simulink model "CLLCTestHarnessPlant"  (R2026a)
settings: Solver=ode23t  StopTime=5e-3  FixedStep=1e-4  MaxStep=1e-6  AbsTol=1e-3
PreLoadFcn:
  | CLLCConverterDefaultInputParameters;
undefined symbols (not defined in the file or in its folder): CLLCCompensator, CLLCController, CLLCDesign, DiscIntNeverNeededParam
libraries: fl_lib x46, nesl_utility x45, ee_lib x35
(part 4 of 4)

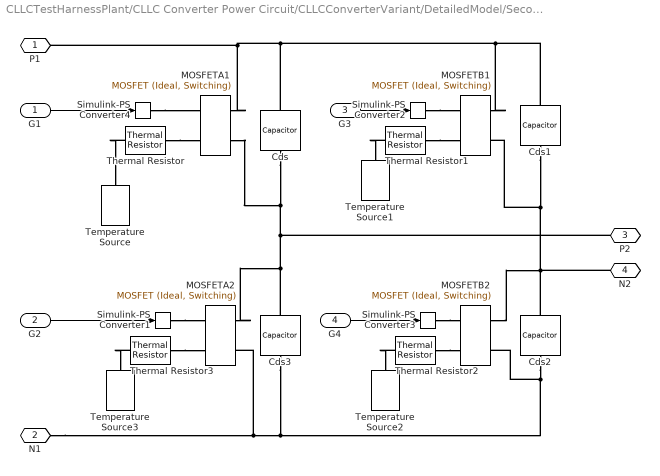
== system CLLCTestHarnessPlant/CLLC Converter Power Circuit/CLLCConverterVariant/DetailedModel/Secondary Converter/Secondary Converter Full Bridge/Ideal MOSFET with Thermal ==
  G1 : Inport
  G2 : Inport  Port=2
  G3 : Inport  Port=3
  G4 : Inport  Port=4
  Cds{,1..3} (4 alike) : fl_lib/Electrical/Electrical Elements/Capacitor  c=SecondaryCparasitic F  r=0.05 Ohm  g=1e-5 1/Ohm  i_specify=off  i_priority=None  i=0 A  i_nominal_specify=off  i_nominal_value=1  i_nominal_unit=A  v_specify=off  v_priority=None  v=0 V  v_nominal_specify=off  v_nominal_value=1  v_nominal_unit=V  vc_specify=on  vc_priority=None  vc=0 V  vc_nominal_specify=off  vc_nominal_value=1  vc_nominal_unit=V
  MOSFETA1 : ee_lib/Semiconductors & Converters/MOSFET (Ideal, Switching)  PartSpecification="{\"CollectionId\":\"MW.SimscapeElectrical\",\"CollectionVersion\":\"1.0.0\",\"DatasetId\":\"Wolfspeed|C3M0015065D|simscape.electrical.mosfetIdealSwitching\",\"DisplayName\":\"Wolfspeed:C3M0015065D\"}"  port_option=ee.enum.controlport.ps  Rds=0.015 % Datasheet derived Ohm  Goff=1.53846153846154e-09 % Datasheet derived S  Vth=2.3 % Datasheet derived V  diode_param=ee.enum.semiconductors.protectionDiode.nodynamics  diode_Vf=1.96 % Datasheet derived V  diode_Ron=0.007 % Wolfspeed XML derived Ohm  diode_Goff=1e-05 % Library default S  diode_C=50e-9 % Parameter not set F  diode_iRM=-235 % Parameter not set A  diode_iF=300 % Parameter not set A  diode_idot=-50 % Parameter not set A/us  diode_trr_param=ee.enum.converters.diodeReverseParam.trr_factor  diode_trr_factor=3 % Parameter not set  diode_trr=15 % Parameter not set us  diode_Qrr=1500 % Parameter not set s*uA  ids_specify=off  ids_priority=None  ids=0 A  ids_nominal_specify=off  ids_nominal_value=1  ids_nominal_unit=A  vds_specify=off  vds_priority=None  vds=0 V  vds_nominal_specify=off  vds_nominal_value=1  vds_nominal_unit=V  vgs_specify=off  vgs_priority=None  vgs=0 V  vgs_nominal_specify=off  vgs_nominal_value=1  vgs_nominal_unit=V  thermal_loss_option=ee.enum.converters.thermalLossOption.tabulated2d  Von_data=[-2.66 -2.44 -1.95 -1.414 -0.78 -0.41 -0.165 -0.082 -0.0343 0 0.037 0.078 0.179 0.43 0.83 1.68 2.597 3.5358 4.01;-2.83 -2.54 -1.975 -1.397 -0.75 -0.38 -0.155 -0.08 -0.03 0 0.034 0.067 0.16 0.39 0.76 1.549 2.4 3.26 3.72;-4.517 -4 -2.934 -1.965 -1 -0.51 -0.2048 -0.1018 -0.041 0 0.042 0.085 0.2 0.496 0.997 2.035 3.12 4.4 5.045;-5 -4.4 -3.2274 -2.1615 -1.1 -0.561 -0.22528 -0.11198 -0.0451 0 0.0462 0.0935 0.22 0.5456 1.0967 2.2385 3.432 4.84 5.5495] % Wolfspeed XML derived V  Tj=[-40 25 175 900] % Wolfspeed XML derived degC  Iout_data=[-225 -200 -150 -100 -50 -25 -10 -5 -2 0 2 5 10 25 50 100 150 200 225] % Wolfspeed XML derived A  tabulateWithVds=true  Eon_data=[0 0.000296720706 0.000619737448 0.001060530449 0.001624353636 0.002289518971 0.003055101185 0.003909744423 0.004857655737;0 0.000278295464 0.000568760601 0.000943163001 0.001425114545 0.001997455958 0.002650659932 0.003379733973 0.004171975428;0 0.000279540051 0.000560708357 0.000946039081 0.001433453185 0.002004053998 0.002654023251 0.00337272687 0.004157099722;0 0.000287359198 0.000590152745 0.001002040365 0.001504786569 0.002087057353 0.002740975089 0.003462716804 0.004216675388;0 0.000330463078 0.000678675657 0.00115234642 0.001730504555 0.002400115956 0.003152121352 0.003982124325 0.004849176696] % Wolfspeed XML derived J  Eoff_data=[0 4.1760829e-05 0.000185261132 0.00041711825 0.000737680365 0.001120556246 0.001567378167 0.002077858914 0.002638540549;0 3.7063976e-05 0.000164368774 0.000376314901 0.000674169231 0.001014162086 0.001431179744 0.001884719714 0.002400774934;0 4.0061697e-05 0.000173404947 0.000400371607 0.000703518786 0.001068777044 0.001494839984 0.001971248404 0.002508087918;0 4.0265683e-05 0.000184357503 0.000417637115 0.000741131352 0.001127026128 0.001573263077 0.002066583681 0.002614125351;0 4.6305536e-05 0.000212011129 0.000480282682 0.000852301054 0.001296080048 0.001809252539 0.002376571234 0.003006244154] % Wolfspeed XML derived J  Eon_data_3D=reshape([0;0;0;0;0;0;0;0;0;0;0;0;0;0;0;0;0;0;0;0;0;0;0;0;0;0;0;0;0;0;0;0;0;0;0;0;0;0;0;0;0;0;0;0;0;0;0;0;0;0;0;0;0;0;0;0;0;0;0;0;0;0;0;0;0;0;0;0;0;0;0;0;0;0;0;0;0;0;0;0;0;0;0;0;0;0;0;0;0;0;0;0;0;0;0;0.000296720706;0.000278295464;0.000279540051;0.000287359198;0.000330463078;0.000619737448;0.000568760601;0.000560708357;0.000590152745;0.000678675657;0.001060530449;0.000943163001;0.000946039081;0.001002040365;0.00115234642;0.001624353636;0.001425114545;0.001433453185;0.001504786569;0.001730504555;0.002289518971;0.001997455958;0.002004053998;0.002087057353;0.002400115956;0.003055101185;0.002650659932;0.002654023251;0.002740975089;0.003152121352;0.003909744423;0.003379733973;0.00337272687;0.003462716804;0.003982124325;0.004857655737;0.004171975428;0.004157099722;0.004216675388;0.004849176696],[5 9 3]) % Wolfspeed XML derived J  Eoff_data_3D=reshape([0;0;0;0;0;0;0;0;0;0;0;0;0;0;0;0;0;0;0;0;0;0;0;0;0;0;0;0;0;0;0;0;0;0;0;0;0;0;0;0;0;0;0;0;0;0;0;0;0;0;0;0;0;0;0;0;0;0;0;0;0;0;0;0;0;0;0;0;0;0;0;0;0;0;0;0;0;0;0;0;0;0;0;0;0;0;0;0;0;0;0;0;0;0;0;4.1760829e-05;3.7063976e-05;4.0061697e-05;4.0265683e-05;4.6305536e-05;0.000185261132;0.000164368774;0.000173404947;0.000184357503;0.000212011129;0.00041711825;0.000376314901;0.000400371607;0.000417637115;0.000480282682;0.000737680365;0.000674169231;0.000703518786;0.000741131352;0.000852301054;0.001120556246;0.001014162086;0.001068777044;0.001127026128;0.001296080048;0.001567378167;0.001431179744;0.001494839984;0.001573263077;0.001809252539;0.002077858914;0.001884719714;0.001971248404;0.002066583681;0.002376571234;0.002638540549;0.002400774934;0.002508087918;0.002614125351;0.003006244154],[5 9 3]) % Wolfspeed XML derived J  Tj_loss=[25 75 125 175 900] % Wolfspeed XML derived degC  Iout_data_loss=[0 13.2 26 38.8 50.8 62.8 74.8 86 97.2] % Wolfspeed XML derived A  Vds_loss=[-10 0 400] % Wolfspeed XML derived V  Eon_scalar=22.86e-3 % Parameter not set J  Eoff_scalar=17.14e-3 % Parameter not set J  Voff=300 % Parameter not set V  Iout_scalar=600 % Parameter not set A  useCurrentFromPreviousCycle=false  useVoltageFromPreviousCycle=false  diodeModelType=ee.enum.converters.diodeModelType.tabulated  diodeTableType=ee.enum.diode.tableType.VfMat  diode_ReverseIVType=ee.enum.diode.diodeReverseIV.constant  diode_IfMat=[.07, .12, .19, 1.75, 4.24, 7.32, 11.2; .16, .3, .72, 2.14, 4.02, 6.35, 9.12] % Parameter not set A  diode_VfMat=[0 2.87 3.94 4.34 5.07 5.76 6.58 7.12 7.53 7.697;0 2.68 3.54 3.9 4.55 5.26 6.12 6.72 7.18 7.38;0 2.31 3.11 3.45 4.06 4.72 5.61 6.24 6.76 6.987;0 2.079 2.799 3.105 3.654 4.248 5.049 5.616 6.084 6.3] % Wolfspeed XML derived V  diode_TjVec=[-40 25 175 900] % Wolfspeed XML derived degC  diode_VfVec=[.5, .7, .9, 1.3, 1.7, 2.1, 2.5] % Parameter not set V  diode_IfVec=[0 0.13 5 10 25 50 100 150 200 225] % Wolfspeed XML derived A  diode_IrMat=[1e-06, 2e-06, 5e-06, 1e-05, 2.5e-05, 5e-05, .0001; 2e-06, 5e-06, 1e-05, 4e-05, 8e-05, .0002, .0005] % Parameter not set A  diode_VrMat=[10, 100, 200, 250, 300, 325, 350; 10, 70, 160, 220, 270, 300, 320] % Parameter not set V  diode_VrVec=[10, 20, 40, 50, 70, 80, 100] % Parameter not set V  diode_IrVec=[1e-06, 2e-06, 5e-06, 1e-05, 2e-05, 5e-05, .0001] % Parameter not set A  diode_Vr=-600 % Parameter not set V  diode_Ls=150 % Parameter not set nH  diode_Erec=0.03 % Parameter not set J  diode_rec_loss_model=ee.enum.diode.reverseRecoveryModelTabulateUpTo3D.fixed  diode_ErecVal=0 % Parameter not set J  diode_scaleWithIandV=false  diode_ErecMat=[0 0;0 0] % Wolfspeed XML derived J  diodeErecMat3D=zeros(2, 3, 2) % Parameter not set J  diode_TjrecVec=[25 35] % Wolfspeed XML derived degC  diode_IfrecVec=[0 10] % Wolfspeed XML derived A  diodeVrecVec=[0, 100] % Parameter not set V  diode_IrecVal=10 % Parameter not set A  diode_VrecVal=10 % Wolfspeed XML derived V  diode_tFilter=1 / 1000 / 100 % Parameter not set s  separateThermalPortForDiode=false  thermal_network_parameterization=ee.enum.thermalNetworkTopology.external  Rth=[.03, .2] % Parameter not set K/W  Rth_Cauer=[0.040544078 0.111521813 0.073003418 0.124838849] % Wolfspeed XML derived K/W  Rth_Foster=[.08, .14, .22, .16] % Parameter not set K/W  thermal_mass_parameterization=ee.enum.thermalNetwork.thermalmass  thermal_mass=[3, 25] % Parameter not set J/K  thermal_mass_Cauer=[0.002121535 0.01054405 0.031037314 0.127325435] % Wolfspeed XML derived J/K  thermal_mass_Foster=[.001, .005, .05, .5] % Parameter not set J/K  thermal_time_constant=[.1, 5] % Parameter not set s  thermal_time_constant_Cauer=[.1, 1, 5] % Parameter not set s  thermal_time_constant_Foster=[7e-05, .0007, .01, .08] % Parameter not set s  thermal_mass_initial_temperatures=[25, 25] % Parameter not set degC  thermal_mass_initial_temperatures_Cauer=[25 25 25 25] % Wolfspeed XML derived degC  junction_thermal_mass=0.1 % Parameter not set J/K  Tvec_initial_Foster=[25, 25, 25, 25] % Parameter not set degC  RthDiode=[.03, .2] % Parameter not set K/W  RthCauerDiode=[0.04054 0.1115 0.073 0.1248] % Wolfspeed XML derived K/W  RthFosterDiode=[.03, .2] % Parameter not set K/W  thermalMassDiode=[3, 25] % Parameter not set J/K  thermalMassCauerDiode=[0.002122 0.01054 0.03104 0.1273] % Wolfspeed XML derived J/K  thermalMassFosterDiode=[33, 50] % Parameter not set J/K  thermalTauDiode=[.1, 5] % Parameter not set s  thermalTauCauerDiode=[.1, 1, 5] % Parameter not set s  thermalTauFosterDiode=[1, 10] % Parameter not set s  thermalMassInitTempDiode=[25, 25] % Parameter not set degC  thermalMassInitTempCauerDiode=[25 25 25 25] % Wolfspeed XML derived degC  junctionthermalMassDiode=0.1 % Parameter not set J/K  TVecInitialFosterDiode=[25, 25, 25, 25] % Parameter not set degC  no_thermal_network=0 % Parameter not set  mosfet_junction_temperature_specify=on  mosfet_junction_temperature_priority=None  mosfet_junction_temperature=SecondarySimTemp_K K  mosfet_junction_temperature_nominal_specify=off  mosfet_junction_temperature_nominal_value=1  mosfet_junction_temperature_nominal_unit=degC  diode_junction_temperature_specify=off  diode_junction_temperature_priority=None  diode_junction_temperature=SecondarySimTemp_K K  diode_junction_temperature_nominal_specify=off  diode_junction_temperature_nominal_value=1  diode_junction_temperature_nominal_unit=degC  Qj_specify=off  Qj_priority=None  Qj=0 W  Qj_nominal_specify=off  Qj_nominal_value=1  Qj_nominal_unit=W  accumulatedSwitchingLosses_specify=off  accumulatedSwitchingLosses_priority=None  accumulatedSwitchingLosses=0 J
      settings: AttributesFormatString=Wolfspeed:C3M0015065D
  MOSFETA2 : ee_lib/Semiconductors & Converters/MOSFET (Ideal, Switching)  PartSpecification="{\"CollectionId\":\"MW.SimscapeElectrical\",\"DatasetId\":\"STMicroelectronics|SCTH35N65G2V-7|simscape.electrical.mosfetIdealSwitching\",\"DisplayName\":\"STMicroelectronics:SCTH35N65G2V-7\"}"  port_option=ee.enum.controlport.ps  Rds=0.015 % Datasheet derived Ohm  Goff=1.53846153846154e-09 % Datasheet derived S  Vth=2.3 % Datasheet derived V  diode_param=ee.enum.semiconductors.protectionDiode.nodynamics  diode_Vf=1.96 % Datasheet derived V  diode_Ron=0.007 % Wolfspeed XML derived Ohm  diode_Goff=1e-05 % Library default S  diode_C=50e-9 % Parameter not set F  diode_iRM=-235 % Parameter not set A  diode_iF=300 % Parameter not set A  diode_idot=-50 % Parameter not set A/us  diode_trr_param=ee.enum.converters.diodeReverseParam.trr_factor  diode_trr_factor=3 % Parameter not set  diode_trr=15 % Parameter not set us  diode_Qrr=1500 % Parameter not set s*uA  ids_specify=off  ids_priority=None  ids=0 A  ids_nominal_specify=off  ids_nominal_value=1  ids_nominal_unit=A  vds_specify=off  vds_priority=None  vds=0 V  vds_nominal_specify=off  vds_nominal_value=1  vds_nominal_unit=V  vgs_specify=off  vgs_priority=None  vgs=0 V  vgs_nominal_specify=off  vgs_nominal_value=1  vgs_nominal_unit=V  thermal_loss_option=ee.enum.converters.thermalLossOption.tabulated2d  Von_data=[-2.66 -2.44 -1.95 -1.414 -0.78 -0.41 -0.165 -0.082 -0.0343 0 0.037 0.078 0.179 0.43 0.83 1.68 2.597 3.5358 4.01;-2.83 -2.54 -1.975 -1.397 -0.75 -0.38 -0.155 -0.08 -0.03 0 0.034 0.067 0.16 0.39 0.76 1.549 2.4 3.26 3.72;-4.517 -4 -2.934 -1.965 -1 -0.51 -0.2048 -0.1018 -0.041 0 0.042 0.085 0.2 0.496 0.997 2.035 3.12 4.4 5.045;-5 -4.4 -3.2274 -2.1615 -1.1 -0.561 -0.22528 -0.11198 -0.0451 0 0.0462 0.0935 0.22 0.5456 1.0967 2.2385 3.432 4.84 5.5495] % Wolfspeed XML derived V  Tj=[-40 25 175 900] % Wolfspeed XML derived degC  Iout_data=[-225 -200 -150 -100 -50 -25 -10 -5 -2 0 2 5 10 25 50 100 150 200 225] % Wolfspeed XML derived A  tabulateWithVds=true  Eon_data=[0 0.000296720706 0.000619737448 0.001060530449 0.001624353636 0.002289518971 0.003055101185 0.003909744423 0.004857655737;0 0.000278295464 0.000568760601 0.000943163001 0.001425114545 0.001997455958 0.002650659932 0.003379733973 0.004171975428;0 0.000279540051 0.000560708357 0.000946039081 0.001433453185 0.002004053998 0.002654023251 0.00337272687 0.004157099722;0 0.000287359198 0.000590152745 0.001002040365 0.001504786569 0.002087057353 0.002740975089 0.003462716804 0.004216675388;0 0.000330463078 0.000678675657 0.00115234642 0.001730504555 0.002400115956 0.003152121352 0.003982124325 0.004849176696] % Wolfspeed XML derived J  Eoff_data=[0 4.1760829e-05 0.000185261132 0.00041711825 0.000737680365 0.001120556246 0.001567378167 0.002077858914 0.002638540549;0 3.7063976e-05 0.000164368774 0.000376314901 0.000674169231 0.001014162086 0.001431179744 0.001884719714 0.002400774934;0 4.0061697e-05 0.000173404947 0.000400371607 0.000703518786 0.001068777044 0.001494839984 0.001971248404 0.002508087918;0 4.0265683e-05 0.000184357503 0.000417637115 0.000741131352 0.001127026128 0.001573263077 0.002066583681 0.002614125351;0 4.6305536e-05 0.000212011129 0.000480282682 0.000852301054 0.001296080048 0.001809252539 0.002376571234 0.003006244154] % Wolfspeed XML derived J  Eon_data_3D=reshape([0;0;0;0;0;0;0;0;0;0;0;0;0;0;0;0;0;0;0;0;0;0;0;0;0;0;0;0;0;0;0;0;0;0;0;0;0;0;0;0;0;0;0;0;0;0;0;0;0;0;0;0;0;0;0;0;0;0;0;0;0;0;0;0;0;0;0;0;0;0;0;0;0;0;0;0;0;0;0;0;0;0;0;0;0;0;0;0;0;0;0;0;0;0;0;0.000296720706;0.000278295464;0.000279540051;0.000287359198;0.000330463078;0.000619737448;0.000568760601;0.000560708357;0.000590152745;0.000678675657;0.001060530449;0.000943163001;0.000946039081;0.001002040365;0.00115234642;0.001624353636;0.001425114545;0.001433453185;0.001504786569;0.001730504555;0.002289518971;0.001997455958;0.002004053998;0.002087057353;0.002400115956;0.003055101185;0.002650659932;0.002654023251;0.002740975089;0.003152121352;0.003909744423;0.003379733973;0.00337272687;0.003462716804;0.003982124325;0.004857655737;0.004171975428;0.004157099722;0.004216675388;0.004849176696],[5 9 3]) % Wolfspeed XML derived J  Eoff_data_3D=reshape([0;0;0;0;0;0;0;0;0;0;0;0;0;0;0;0;0;0;0;0;0;0;0;0;0;0;0;0;0;0;0;0;0;0;0;0;0;0;0;0;0;0;0;0;0;0;0;0;0;0;0;0;0;0;0;0;0;0;0;0;0;0;0;0;0;0;0;0;0;0;0;0;0;0;0;0;0;0;0;0;0;0;0;0;0;0;0;0;0;0;0;0;0;0;0;4.1760829e-05;3.7063976e-05;4.0061697e-05;4.0265683e-05;4.6305536e-05;0.000185261132;0.000164368774;0.000173404947;0.000184357503;0.000212011129;0.00041711825;0.000376314901;0.000400371607;0.000417637115;0.000480282682;0.000737680365;0.000674169231;0.000703518786;0.000741131352;0.000852301054;0.001120556246;0.001014162086;0.001068777044;0.001127026128;0.001296080048;0.001567378167;0.001431179744;0.001494839984;0.001573263077;0.001809252539;0.002077858914;0.001884719714;0.001971248404;0.002066583681;0.002376571234;0.002638540549;0.002400774934;0.002508087918;0.002614125351;0.003006244154],[5 9 3]) % Wolfspeed XML derived J  Tj_loss=[25 75 125 175 900] % Wolfspeed XML derived degC  Iout_data_loss=[0 13.2 26 38.8 50.8 62.8 74.8 86 97.2] % Wolfspeed XML derived A  Vds_loss=[-10 0 400] % Wolfspeed XML derived V  Eon_scalar=22.86e-3 % Parameter not set J  Eoff_scalar=17.14e-3 % Parameter not set J  Voff=300 % Parameter not set V  Iout_scalar=600 % Parameter not set A  useCurrentFromPreviousCycle=false  useVoltageFromPreviousCycle=false  diodeModelType=ee.enum.converters.diodeModelType.tabulated  diodeTableType=ee.enum.diode.tableType.VfMat  diode_ReverseIVType=ee.enum.diode.diodeReverseIV.constant  diode_IfMat=[.07, .12, .19, 1.75, 4.24, 7.32, 11.2; .16, .3, .72, 2.14, 4.02, 6.35, 9.12] % Parameter not set A  diode_VfMat=[0 2.87 3.94 4.34 5.07 5.76 6.58 7.12 7.53 7.697;0 2.68 3.54 3.9 4.55 5.26 6.12 6.72 7.18 7.38;0 2.31 3.11 3.45 4.06 4.72 5.61 6.24 6.76 6.987;0 2.079 2.799 3.105 3.654 4.248 5.049 5.616 6.084 6.3] % Wolfspeed XML derived V  diode_TjVec=[-40 25 175 900] % Wolfspeed XML derived degC  diode_VfVec=[.5, .7, .9, 1.3, 1.7, 2.1, 2.5] % Parameter not set V  diode_IfVec=[0 0.13 5 10 25 50 100 150 200 225] % Wolfspeed XML derived A  diode_IrMat=[1e-06, 2e-06, 5e-06, 1e-05, 2.5e-05, 5e-05, .0001; 2e-06, 5e-06, 1e-05, 4e-05, 8e-05, .0002, .0005] % Parameter not set A  diode_VrMat=[10, 100, 200, 250, 300, 325, 350; 10, 70, 160, 220, 270, 300, 320] % Parameter not set V  diode_VrVec=[10, 20, 40, 50, 70, 80, 100] % Parameter not set V  diode_IrVec=[1e-06, 2e-06, 5e-06, 1e-05, 2e-05, 5e-05, .0001] % Parameter not set A  diode_Vr=-600 % Parameter not set V  diode_Ls=150 % Parameter not set nH  diode_Erec=0.03 % Parameter not set J  diode_rec_loss_model=ee.enum.diode.reverseRecoveryModelTabulateUpTo3D.fixed  diode_ErecVal=0 % Parameter not set J  diode_scaleWithIandV=false  diode_ErecMat=[0 0;0 0] % Wolfspeed XML derived J  diodeErecMat3D=zeros(2, 3, 2) % Parameter not set J  diode_TjrecVec=[25 35] % Wolfspeed XML derived degC  diode_IfrecVec=[0 10] % Wolfspeed XML derived A  diodeVrecVec=[0, 100] % Parameter not set V  diode_IrecVal=10 % Parameter not set A  diode_VrecVal=10 % Wolfspeed XML derived V  diode_tFilter=1 / 1000 / 100 % Parameter not set s  separateThermalPortForDiode=false  thermal_network_parameterization=ee.enum.thermalNetworkTopology.external  Rth=[.03, .2] % Parameter not set K/W  Rth_Cauer=[0.040544078 0.111521813 0.073003418 0.124838849] % Wolfspeed XML derived K/W  Rth_Foster=[.08, .14, .22, .16] % Parameter not set K/W  thermal_mass_parameterization=ee.enum.thermalNetwork.thermalmass  thermal_mass=[3, 25] % Parameter not set J/K  thermal_mass_Cauer=[0.002121535 0.01054405 0.031037314 0.127325435] % Wolfspeed XML derived J/K  thermal_mass_Foster=[.001, .005, .05, .5] % Parameter not set J/K  thermal_time_constant=[.1, 5] % Parameter not set s  thermal_time_constant_Cauer=[.1, 1, 5] % Parameter not set s  thermal_time_constant_Foster=[7e-05, .0007, .01, .08] % Parameter not set s  thermal_mass_initial_temperatures=[25, 25] % Parameter not set degC  thermal_mass_initial_temperatures_Cauer=[25 25 25 25] % Wolfspeed XML derived degC  junction_thermal_mass=0.1 % Parameter not set J/K  Tvec_initial_Foster=[25, 25, 25, 25] % Parameter not set degC  RthDiode=[.03, .2] % Parameter not set K/W  RthCauerDiode=[0.04054 0.1115 0.073 0.1248] % Wolfspeed XML derived K/W  RthFosterDiode=[.03, .2] % Parameter not set K/W  thermalMassDiode=[3, 25] % Parameter not set J/K  thermalMassCauerDiode=[0.002122 0.01054 0.03104 0.1273] % Wolfspeed XML derived J/K  thermalMassFosterDiode=[33, 50] % Parameter not set J/K  thermalTauDiode=[.1, 5] % Parameter not set s  thermalTauCauerDiode=[.1, 1, 5] % Parameter not set s  thermalTauFosterDiode=[1, 10] % Parameter not set s  thermalMassInitTempDiode=[25, 25] % Parameter not set degC  thermalMassInitTempCauerDiode=[25 25 25 25] % Wolfspeed XML derived degC  junctionthermalMassDiode=0.1 % Parameter not set J/K  TVecInitialFosterDiode=[25, 25, 25, 25] % Parameter not set degC  no_thermal_network=0 % Parameter not set  mosfet_junction_temperature_specify=on  mosfet_junction_temperature_priority=None  mosfet_junction_temperature=SecondarySimTemp_K K  mosfet_junction_temperature_nominal_specify=off  mosfet_junction_temperature_nominal_value=1  mosfet_junction_temperature_nominal_unit=degC  diode_junction_temperature_specify=off  diode_junction_temperature_priority=None  diode_junction_temperature=SecondarySimTemp_K K  diode_junction_temperature_nominal_specify=off  diode_junction_temperature_nominal_value=1  diode_junction_temperature_nominal_unit=degC  Qj_specify=off  Qj_priority=None  Qj=0 W  Qj_nominal_specify=off  Qj_nominal_value=1  Qj_nominal_unit=W  accumulatedSwitchingLosses_specify=off  accumulatedSwitchingLosses_priority=None  accumulatedSwitchingLosses=0 J
      settings: AttributesFormatString=STMicroelectronics:SCTH35N65G2V-7
  MOSFETB1 : ee_lib/Semiconductors & Converters/MOSFET (Ideal, Switching)  PartSpecification="{\"CollectionId\":\"MW.SimscapeElectrical\",\"DatasetId\":\"STMicroelectronics|SCTH35N65G2V-7|simscape.electrical.mosfetIdealSwitching\",\"DisplayName\":\"STMicroelectronics:SCTH35N65G2V-7\"}"  port_option=ee.enum.controlport.ps  Rds=0.015 % Datasheet derived Ohm  Goff=1.53846153846154e-09 % Datasheet derived S  Vth=2.3 % Datasheet derived V  diode_param=ee.enum.semiconductors.protectionDiode.nodynamics  diode_Vf=1.96 % Datasheet derived V  diode_Ron=0.007 % Wolfspeed XML derived Ohm  diode_Goff=1e-05 % Library default S  diode_C=50e-9 % Parameter not set F  diode_iRM=-235 % Parameter not set A  diode_iF=300 % Parameter not set A  diode_idot=-50 % Parameter not set A/us  diode_trr_param=ee.enum.converters.diodeReverseParam.trr_factor  diode_trr_factor=3 % Parameter not set  diode_trr=15 % Parameter not set us  diode_Qrr=1500 % Parameter not set s*uA  ids_specify=off  ids_priority=None  ids=0 A  ids_nominal_specify=off  ids_nominal_value=1  ids_nominal_unit=A  vds_specify=off  vds_priority=None  vds=0 V  vds_nominal_specify=off  vds_nominal_value=1  vds_nominal_unit=V  vgs_specify=off  vgs_priority=None  vgs=0 V  vgs_nominal_specify=off  vgs_nominal_value=1  vgs_nominal_unit=V  thermal_loss_option=ee.enum.converters.thermalLossOption.tabulated2d  Von_data=[-2.66 -2.44 -1.95 -1.414 -0.78 -0.41 -0.165 -0.082 -0.0343 0 0.037 0.078 0.179 0.43 0.83 1.68 2.597 3.5358 4.01;-2.83 -2.54 -1.975 -1.397 -0.75 -0.38 -0.155 -0.08 -0.03 0 0.034 0.067 0.16 0.39 0.76 1.549 2.4 3.26 3.72;-4.517 -4 -2.934 -1.965 -1 -0.51 -0.2048 -0.1018 -0.041 0 0.042 0.085 0.2 0.496 0.997 2.035 3.12 4.4 5.045;-5 -4.4 -3.2274 -2.1615 -1.1 -0.561 -0.22528 -0.11198 -0.0451 0 0.0462 0.0935 0.22 0.5456 1.0967 2.2385 3.432 4.84 5.5495] % Wolfspeed XML derived V  Tj=[-40 25 175 900] % Wolfspeed XML derived degC  Iout_data=[-225 -200 -150 -100 -50 -25 -10 -5 -2 0 2 5 10 25 50 100 150 200 225] % Wolfspeed XML derived A  tabulateWithVds=true  Eon_data=[0 0.000296720706 0.000619737448 0.001060530449 0.001624353636 0.002289518971 0.003055101185 0.003909744423 0.004857655737;0 0.000278295464 0.000568760601 0.000943163001 0.001425114545 0.001997455958 0.002650659932 0.003379733973 0.004171975428;0 0.000279540051 0.000560708357 0.000946039081 0.001433453185 0.002004053998 0.002654023251 0.00337272687 0.004157099722;0 0.000287359198 0.000590152745 0.001002040365 0.001504786569 0.002087057353 0.002740975089 0.003462716804 0.004216675388;0 0.000330463078 0.000678675657 0.00115234642 0.001730504555 0.002400115956 0.003152121352 0.003982124325 0.004849176696] % Wolfspeed XML derived J  Eoff_data=[0 4.1760829e-05 0.000185261132 0.00041711825 0.000737680365 0.001120556246 0.001567378167 0.002077858914 0.002638540549;0 3.7063976e-05 0.000164368774 0.000376314901 0.000674169231 0.001014162086 0.001431179744 0.001884719714 0.002400774934;0 4.0061697e-05 0.000173404947 0.000400371607 0.000703518786 0.001068777044 0.001494839984 0.001971248404 0.002508087918;0 4.0265683e-05 0.000184357503 0.000417637115 0.000741131352 0.001127026128 0.001573263077 0.002066583681 0.002614125351;0 4.6305536e-05 0.000212011129 0.000480282682 0.000852301054 0.001296080048 0.001809252539 0.002376571234 0.003006244154] % Wolfspeed XML derived J  Eon_data_3D=reshape([0;0;0;0;0;0;0;0;0;0;0;0;0;0;0;0;0;0;0;0;0;0;0;0;0;0;0;0;0;0;0;0;0;0;0;0;0;0;0;0;0;0;0;0;0;0;0;0;0;0;0;0;0;0;0;0;0;0;0;0;0;0;0;0;0;0;0;0;0;0;0;0;0;0;0;0;0;0;0;0;0;0;0;0;0;0;0;0;0;0;0;0;0;0;0;0.000296720706;0.000278295464;0.000279540051;0.000287359198;0.000330463078;0.000619737448;0.000568760601;0.000560708357;0.000590152745;0.000678675657;0.001060530449;0.000943163001;0.000946039081;0.001002040365;0.00115234642;0.001624353636;0.001425114545;0.001433453185;0.001504786569;0.001730504555;0.002289518971;0.001997455958;0.002004053998;0.002087057353;0.002400115956;0.003055101185;0.002650659932;0.002654023251;0.002740975089;0.003152121352;0.003909744423;0.003379733973;0.00337272687;0.003462716804;0.003982124325;0.004857655737;0.004171975428;0.004157099722;0.004216675388;0.004849176696],[5 9 3]) % Wolfspeed XML derived J  Eoff_data_3D=reshape([0;0;0;0;0;0;0;0;0;0;0;0;0;0;0;0;0;0;0;0;0;0;0;0;0;0;0;0;0;0;0;0;0;0;0;0;0;0;0;0;0;0;0;0;0;0;0;0;0;0;0;0;0;0;0;0;0;0;0;0;0;0;0;0;0;0;0;0;0;0;0;0;0;0;0;0;0;0;0;0;0;0;0;0;0;0;0;0;0;0;0;0;0;0;0;4.1760829e-05;3.7063976e-05;4.0061697e-05;4.0265683e-05;4.6305536e-05;0.000185261132;0.000164368774;0.000173404947;0.000184357503;0.000212011129;0.00041711825;0.000376314901;0.000400371607;0.000417637115;0.000480282682;0.000737680365;0.000674169231;0.000703518786;0.000741131352;0.000852301054;0.001120556246;0.001014162086;0.001068777044;0.001127026128;0.001296080048;0.001567378167;0.001431179744;0.001494839984;0.001573263077;0.001809252539;0.002077858914;0.001884719714;0.001971248404;0.002066583681;0.002376571234;0.002638540549;0.002400774934;0.002508087918;0.002614125351;0.003006244154],[5 9 3]) % Wolfspeed XML derived J  Tj_loss=[25 75 125 175 900] % Wolfspeed XML derived degC  Iout_data_loss=[0 13.2 26 38.8 50.8 62.8 74.8 86 97.2] % Wolfspeed XML derived A  Vds_loss=[-10 0 400] % Wolfspeed XML derived V  Eon_scalar=22.86e-3 % Parameter not set J  Eoff_scalar=17.14e-3 % Parameter not set J  Voff=300 % Parameter not set V  Iout_scalar=600 % Parameter not set A  useCurrentFromPreviousCycle=false  useVoltageFromPreviousCycle=false  diodeModelType=ee.enum.converters.diodeModelType.tabulated  diodeTableType=ee.enum.diode.tableType.VfMat  diode_ReverseIVType=ee.enum.diode.diodeReverseIV.constant  diode_IfMat=[.07, .12, .19, 1.75, 4.24, 7.32, 11.2; .16, .3, .72, 2.14, 4.02, 6.35, 9.12] % Parameter not set A  diode_VfMat=[0 2.87 3.94 4.34 5.07 5.76 6.58 7.12 7.53 7.697;0 2.68 3.54 3.9 4.55 5.26 6.12 6.72 7.18 7.38;0 2.31 3.11 3.45 4.06 4.72 5.61 6.24 6.76 6.987;0 2.079 2.799 3.105 3.654 4.248 5.049 5.616 6.084 6.3] % Wolfspeed XML derived V  diode_TjVec=[-40 25 175 900] % Wolfspeed XML derived degC  diode_VfVec=[.5, .7, .9, 1.3, 1.7, 2.1, 2.5] % Parameter not set V  diode_IfVec=[0 0.13 5 10 25 50 100 150 200 225] % Wolfspeed XML derived A  diode_IrMat=[1e-06, 2e-06, 5e-06, 1e-05, 2.5e-05, 5e-05, .0001; 2e-06, 5e-06, 1e-05, 4e-05, 8e-05, .0002, .0005] % Parameter not set A  diode_VrMat=[10, 100, 200, 250, 300, 325, 350; 10, 70, 160, 220, 270, 300, 320] % Parameter not set V  diode_VrVec=[10, 20, 40, 50, 70, 80, 100] % Parameter not set V  diode_IrVec=[1e-06, 2e-06, 5e-06, 1e-05, 2e-05, 5e-05, .0001] % Parameter not set A  diode_Vr=-600 % Parameter not set V  diode_Ls=150 % Parameter not set nH  diode_Erec=0.03 % Parameter not set J  diode_rec_loss_model=ee.enum.diode.reverseRecoveryModelTabulateUpTo3D.fixed  diode_ErecVal=0 % Parameter not set J  diode_scaleWithIandV=false  diode_ErecMat=[0 0;0 0] % Wolfspeed XML derived J  diodeErecMat3D=zeros(2, 3, 2) % Parameter not set J  diode_TjrecVec=[25 35] % Wolfspeed XML derived degC  diode_IfrecVec=[0 10] % Wolfspeed XML derived A  diodeVrecVec=[0, 100] % Parameter not set V  diode_IrecVal=10 % Parameter not set A  diode_VrecVal=10 % Wolfspeed XML derived V  diode_tFilter=1 / 1000 / 100 % Parameter not set s  separateThermalPortForDiode=false  thermal_network_parameterization=ee.enum.thermalNetworkTopology.external  Rth=[.03, .2] % Parameter not set K/W  Rth_Cauer=[0.040544078 0.111521813 0.073003418 0.124838849] % Wolfspeed XML derived K/W  Rth_Foster=[.08, .14, .22, .16] % Parameter not set K/W  thermal_mass_parameterization=ee.enum.thermalNetwork.thermalmass  thermal_mass=[3, 25] % Parameter not set J/K  thermal_mass_Cauer=[0.002121535 0.01054405 0.031037314 0.127325435] % Wolfspeed XML derived J/K  thermal_mass_Foster=[.001, .005, .05, .5] % Parameter not set J/K  thermal_time_constant=[.1, 5] % Parameter not set s  thermal_time_constant_Cauer=[.1, 1, 5] % Parameter not set s  thermal_time_constant_Foster=[7e-05, .0007, .01, .08] % Parameter not set s  thermal_mass_initial_temperatures=[25, 25] % Parameter not set degC  thermal_mass_initial_temperatures_Cauer=[25 25 25 25] % Wolfspeed XML derived degC  junction_thermal_mass=0.1 % Parameter not set J/K  Tvec_initial_Foster=[25, 25, 25, 25] % Parameter not set degC  RthDiode=[.03, .2] % Parameter not set K/W  RthCauerDiode=[0.04054 0.1115 0.073 0.1248] % Wolfspeed XML derived K/W  RthFosterDiode=[.03, .2] % Parameter not set K/W  thermalMassDiode=[3, 25] % Parameter not set J/K  thermalMassCauerDiode=[0.002122 0.01054 0.03104 0.1273] % Wolfspeed XML derived J/K  thermalMassFosterDiode=[33, 50] % Parameter not set J/K  thermalTauDiode=[.1, 5] % Parameter not set s  thermalTauCauerDiode=[.1, 1, 5] % Parameter not set s  thermalTauFosterDiode=[1, 10] % Parameter not set s  thermalMassInitTempDiode=[25, 25] % Parameter not set degC  thermalMassInitTempCauerDiode=[25 25 25 25] % Wolfspeed XML derived degC  junctionthermalMassDiode=0.1 % Parameter not set J/K  TVecInitialFosterDiode=[25, 25, 25, 25] % Parameter not set degC  no_thermal_network=0 % Parameter not set  mosfet_junction_temperature_specify=on  mosfet_junction_temperature_priority=None  mosfet_junction_temperature=SecondarySimTemp_K K  mosfet_junction_temperature_nominal_specify=off  mosfet_junction_temperature_nominal_value=1  mosfet_junction_temperature_nominal_unit=degC  diode_junction_temperature_specify=off  diode_junction_temperature_priority=None  diode_junction_temperature=SecondarySimTemp_K K  diode_junction_temperature_nominal_specify=off  diode_junction_temperature_nominal_value=1  diode_junction_temperature_nominal_unit=degC  Qj_specify=off  Qj_priority=None  Qj=0 W  Qj_nominal_specify=off  Qj_nominal_value=1  Qj_nominal_unit=W  accumulatedSwitchingLosses_specify=off  accumulatedSwitchingLosses_priority=None  accumulatedSwitchingLosses=0 J
      settings: AttributesFormatString=STMicroelectronics:SCTH35N65G2V-7
  MOSFETB2 : ee_lib/Semiconductors & Converters/MOSFET (Ideal, Switching)  PartSpecification="{\"CollectionId\":\"MW.SimscapeElectrical\",\"DatasetId\":\"STMicroelectronics|SCTH35N65G2V-7|simscape.electrical.mosfetIdealSwitching\",\"DisplayName\":\"STMicroelectronics:SCTH35N65G2V-7\"}"  port_option=ee.enum.controlport.ps  Rds=0.015 % Datasheet derived Ohm  Goff=1.53846153846154e-09 % Datasheet derived S  Vth=2.3 % Datasheet derived V  diode_param=ee.enum.semiconductors.protectionDiode.nodynamics  diode_Vf=1.96 % Datasheet derived V  diode_Ron=0.007 % Wolfspeed XML derived Ohm  diode_Goff=1e-05 % Library default S  diode_C=50e-9 % Parameter not set F  diode_iRM=-235 % Parameter not set A  diode_iF=300 % Parameter not set A  diode_idot=-50 % Parameter not set A/us  diode_trr_param=ee.enum.converters.diodeReverseParam.trr_factor  diode_trr_factor=3 % Parameter not set  diode_trr=15 % Parameter not set us  diode_Qrr=1500 % Parameter not set s*uA  ids_specify=off  ids_priority=None  ids=0 A  ids_nominal_specify=off  ids_nominal_value=1  ids_nominal_unit=A  vds_specify=off  vds_priority=None  vds=0 V  vds_nominal_specify=off  vds_nominal_value=1  vds_nominal_unit=V  vgs_specify=off  vgs_priority=None  vgs=0 V  vgs_nominal_specify=off  vgs_nominal_value=1  vgs_nominal_unit=V  thermal_loss_option=ee.enum.converters.thermalLossOption.tabulated2d  Von_data=[-2.66 -2.44 -1.95 -1.414 -0.78 -0.41 -0.165 -0.082 -0.0343 0 0.037 0.078 0.179 0.43 0.83 1.68 2.597 3.5358 4.01;-2.83 -2.54 -1.975 -1.397 -0.75 -0.38 -0.155 -0.08 -0.03 0 0.034 0.067 0.16 0.39 0.76 1.549 2.4 3.26 3.72;-4.517 -4 -2.934 -1.965 -1 -0.51 -0.2048 -0.1018 -0.041 0 0.042 0.085 0.2 0.496 0.997 2.035 3.12 4.4 5.045;-5 -4.4 -3.2274 -2.1615 -1.1 -0.561 -0.22528 -0.11198 -0.0451 0 0.0462 0.0935 0.22 0.5456 1.0967 2.2385 3.432 4.84 5.5495] % Wolfspeed XML derived V  Tj=[-40 25 175 900] % Wolfspeed XML derived degC  Iout_data=[-225 -200 -150 -100 -50 -25 -10 -5 -2 0 2 5 10 25 50 100 150 200 225] % Wolfspeed XML derived A  tabulateWithVds=true  Eon_data=[0 0.000296720706 0.000619737448 0.001060530449 0.001624353636 0.002289518971 0.003055101185 0.003909744423 0.004857655737;0 0.000278295464 0.000568760601 0.000943163001 0.001425114545 0.001997455958 0.002650659932 0.003379733973 0.004171975428;0 0.000279540051 0.000560708357 0.000946039081 0.001433453185 0.002004053998 0.002654023251 0.00337272687 0.004157099722;0 0.000287359198 0.000590152745 0.001002040365 0.001504786569 0.002087057353 0.002740975089 0.003462716804 0.004216675388;0 0.000330463078 0.000678675657 0.00115234642 0.001730504555 0.002400115956 0.003152121352 0.003982124325 0.004849176696] % Wolfspeed XML derived J  Eoff_data=[0 4.1760829e-05 0.000185261132 0.00041711825 0.000737680365 0.001120556246 0.001567378167 0.002077858914 0.002638540549;0 3.7063976e-05 0.000164368774 0.000376314901 0.000674169231 0.001014162086 0.001431179744 0.001884719714 0.002400774934;0 4.0061697e-05 0.000173404947 0.000400371607 0.000703518786 0.001068777044 0.001494839984 0.001971248404 0.002508087918;0 4.0265683e-05 0.000184357503 0.000417637115 0.000741131352 0.001127026128 0.001573263077 0.002066583681 0.002614125351;0 4.6305536e-05 0.000212011129 0.000480282682 0.000852301054 0.001296080048 0.001809252539 0.002376571234 0.003006244154] % Wolfspeed XML derived J  Eon_data_3D=reshape([0;0;0;0;0;0;0;0;0;0;0;0;0;0;0;0;0;0;0;0;0;0;0;0;0;0;0;0;0;0;0;0;0;0;0;0;0;0;0;0;0;0;0;0;0;0;0;0;0;0;0;0;0;0;0;0;0;0;0;0;0;0;0;0;0;0;0;0;0;0;0;0;0;0;0;0;0;0;0;0;0;0;0;0;0;0;0;0;0;0;0;0;0;0;0;0.000296720706;0.000278295464;0.000279540051;0.000287359198;0.000330463078;0.000619737448;0.000568760601;0.000560708357;0.000590152745;0.000678675657;0.001060530449;0.000943163001;0.000946039081;0.001002040365;0.00115234642;0.001624353636;0.001425114545;0.001433453185;0.001504786569;0.001730504555;0.002289518971;0.001997455958;0.002004053998;0.002087057353;0.002400115956;0.003055101185;0.002650659932;0.002654023251;0.002740975089;0.003152121352;0.003909744423;0.003379733973;0.00337272687;0.003462716804;0.003982124325;0.004857655737;0.004171975428;0.004157099722;0.004216675388;0.004849176696],[5 9 3]) % Wolfspeed XML derived J  Eoff_data_3D=reshape([0;0;0;0;0;0;0;0;0;0;0;0;0;0;0;0;0;0;0;0;0;0;0;0;0;0;0;0;0;0;0;0;0;0;0;0;0;0;0;0;0;0;0;0;0;0;0;0;0;0;0;0;0;0;0;0;0;0;0;0;0;0;0;0;0;0;0;0;0;0;0;0;0;0;0;0;0;0;0;0;0;0;0;0;0;0;0;0;0;0;0;0;0;0;0;4.1760829e-05;3.7063976e-05;4.0061697e-05;4.0265683e-05;4.6305536e-05;0.000185261132;0.000164368774;0.000173404947;0.000184357503;0.000212011129;0.00041711825;0.000376314901;0.000400371607;0.000417637115;0.000480282682;0.000737680365;0.000674169231;0.000703518786;0.000741131352;0.000852301054;0.001120556246;0.001014162086;0.001068777044;0.001127026128;0.001296080048;0.001567378167;0.001431179744;0.001494839984;0.001573263077;0.001809252539;0.002077858914;0.001884719714;0.001971248404;0.002066583681;0.002376571234;0.002638540549;0.002400774934;0.002508087918;0.002614125351;0.003006244154],[5 9 3]) % Wolfspeed XML derived J  Tj_loss=[25 75 125 175 900] % Wolfspeed XML derived degC  Iout_data_loss=[0 13.2 26 38.8 50.8 62.8 74.8 86 97.2] % Wolfspeed XML derived A  Vds_loss=[-10 0 400] % Wolfspeed XML derived V  Eon_scalar=22.86e-3 % Parameter not set J  Eoff_scalar=17.14e-3 % Parameter not set J  Voff=300 % Parameter not set V  Iout_scalar=600 % Parameter not set A  useCurrentFromPreviousCycle=false  useVoltageFromPreviousCycle=false  diodeModelType=ee.enum.converters.diodeModelType.tabulated  diodeTableType=ee.enum.diode.tableType.VfMat  diode_ReverseIVType=ee.enum.diode.diodeReverseIV.constant  diode_IfMat=[.07, .12, .19, 1.75, 4.24, 7.32, 11.2; .16, .3, .72, 2.14, 4.02, 6.35, 9.12] % Parameter not set A  diode_VfMat=[0 2.87 3.94 4.34 5.07 5.76 6.58 7.12 7.53 7.697;0 2.68 3.54 3.9 4.55 5.26 6.12 6.72 7.18 7.38;0 2.31 3.11 3.45 4.06 4.72 5.61 6.24 6.76 6.987;0 2.079 2.799 3.105 3.654 4.248 5.049 5.616 6.084 6.3] % Wolfspeed XML derived V  diode_TjVec=[-40 25 175 900] % Wolfspeed XML derived degC  diode_VfVec=[.5, .7, .9, 1.3, 1.7, 2.1, 2.5] % Parameter not set V  diode_IfVec=[0 0.13 5 10 25 50 100 150 200 225] % Wolfspeed XML derived A  diode_IrMat=[1e-06, 2e-06, 5e-06, 1e-05, 2.5e-05, 5e-05, .0001; 2e-06, 5e-06, 1e-05, 4e-05, 8e-05, .0002, .0005] % Parameter not set A  diode_VrMat=[10, 100, 200, 250, 300, 325, 350; 10, 70, 160, 220, 270, 300, 320] % Parameter not set V  diode_VrVec=[10, 20, 40, 50, 70, 80, 100] % Parameter not set V  diode_IrVec=[1e-06, 2e-06, 5e-06, 1e-05, 2e-05, 5e-05, .0001] % Parameter not set A  diode_Vr=-600 % Parameter not set V  diode_Ls=150 % Parameter not set nH  diode_Erec=0.03 % Parameter not set J  diode_rec_loss_model=ee.enum.diode.reverseRecoveryModelTabulateUpTo3D.fixed  diode_ErecVal=0 % Parameter not set J  diode_scaleWithIandV=false  diode_ErecMat=[0 0;0 0] % Wolfspeed XML derived J  diodeErecMat3D=zeros(2, 3, 2) % Parameter not set J  diode_TjrecVec=[25 35] % Wolfspeed XML derived degC  diode_IfrecVec=[0 10] % Wolfspeed XML derived A  diodeVrecVec=[0, 100] % Parameter not set V  diode_IrecVal=10 % Parameter not set A  diode_VrecVal=10 % Wolfspeed XML derived V  diode_tFilter=1 / 1000 / 100 % Parameter not set s  separateThermalPortForDiode=false  thermal_network_parameterization=ee.enum.thermalNetworkTopology.external  Rth=[.03, .2] % Parameter not set K/W  Rth_Cauer=[0.040544078 0.111521813 0.073003418 0.124838849] % Wolfspeed XML derived K/W  Rth_Foster=[.08, .14, .22, .16] % Parameter not set K/W  thermal_mass_parameterization=ee.enum.thermalNetwork.thermalmass  thermal_mass=[3, 25] % Parameter not set J/K  thermal_mass_Cauer=[0.002121535 0.01054405 0.031037314 0.127325435] % Wolfspeed XML derived J/K  thermal_mass_Foster=[.001, .005, .05, .5] % Parameter not set J/K  thermal_time_constant=[.1, 5] % Parameter not set s  thermal_time_constant_Cauer=[.1, 1, 5] % Parameter not set s  thermal_time_constant_Foster=[7e-05, .0007, .01, .08] % Parameter not set s  thermal_mass_initial_temperatures=[25, 25] % Parameter not set degC  thermal_mass_initial_temperatures_Cauer=[25 25 25 25] % Wolfspeed XML derived degC  junction_thermal_mass=0.1 % Parameter not set J/K  Tvec_initial_Foster=[25, 25, 25, 25] % Parameter not set degC  RthDiode=[.03, .2] % Parameter not set K/W  RthCauerDiode=[0.04054 0.1115 0.073 0.1248] % Wolfspeed XML derived K/W  RthFosterDiode=[.03, .2] % Parameter not set K/W  thermalMassDiode=[3, 25] % Parameter not set J/K  thermalMassCauerDiode=[0.002122 0.01054 0.03104 0.1273] % Wolfspeed XML derived J/K  thermalMassFosterDiode=[33, 50] % Parameter not set J/K  thermalTauDiode=[.1, 5] % Parameter not set s  thermalTauCauerDiode=[.1, 1, 5] % Parameter not set s  thermalTauFosterDiode=[1, 10] % Parameter not set s  thermalMassInitTempDiode=[25, 25] % Parameter not set degC  thermalMassInitTempCauerDiode=[25 25 25 25] % Wolfspeed XML derived degC  junctionthermalMassDiode=0.1 % Parameter not set J/K  TVecInitialFosterDiode=[25, 25, 25, 25] % Parameter not set degC  no_thermal_network=0 % Parameter not set  mosfet_junction_temperature_specify=on  mosfet_junction_temperature_priority=None  mosfet_junction_temperature=SecondarySimTemp_K K  mosfet_junction_temperature_nominal_specify=off  mosfet_junction_temperature_nominal_value=1  mosfet_junction_temperature_nominal_unit=degC  diode_junction_temperature_specify=off  diode_junction_temperature_priority=None  diode_junction_temperature=SecondarySimTemp_K K  diode_junction_temperature_nominal_specify=off  diode_junction_temperature_nominal_value=1  diode_junction_temperature_nominal_unit=degC  Qj_specify=off  Qj_priority=None  Qj=0 W  Qj_nominal_specify=off  Qj_nominal_value=1  Qj_nominal_unit=W  accumulatedSwitchingLosses_specify=off  accumulatedSwitchingLosses_priority=None  accumulatedSwitchingLosses=0 J
      settings: AttributesFormatString=STMicroelectronics:SCTH35N65G2V-7
  Simulink-PS Converter{1..4} (4 alike) : nesl_utility/Simulink-PS Converter  PhysicalDomain=network_engine_domain  SubClassName=ps_input  LeftPortType=input  RightPortType=output  PseudoPeriodic=off  Frequencies=[]  NoiseDistribution=none  NoiseParameters=[]  Unit=1  AffineConversion=off  FilteringAndDerivatives=provide  SimscapeFilterOrder=1  InputFilterTimeConstant=0.001  UdotUserProvided=0
  Temperature Source{,1..3} (4 alike) : fl_lib/Thermal/Thermal Sources/Temperature Source  temperature=SecondarySimTemp_K K
  Thermal Resistor{,1..3} (4 alike) : ee_lib/Passive/Thermal/Thermal Resistor  R=1e-4 K/W  T_specify=on  T_priority=None  T=0 K  T_nominal_specify=off  T_nominal_value=1  T_nominal_unit=K  Q_specify=off  Q_priority=None  Q=0 W  Q_nominal_specify=off  Q_nominal_value=1  Q_nominal_unit=W
  P1 : PMIOPort  Side=Right
  N1 : PMIOPort  Port=2  Side=Right
  P2 : PMIOPort  Port=3  Side=Left
  N2 : PMIOPort  Port=4  Side=Left
  wires:
  G1/1 -> Simulink-PS Converter4/1
  G3/1 -> Simulink-PS Converter2/1
  G4/1 -> Simulink-PS Converter3/1
  G2/1 -> Simulink-PS Converter1/1
  connections:
  P1/RConn1 -- MOSFETB1/RConn1 -- Cds1/LConn1 -- Cds/LConn1 -- MOSFETA1/RConn1
  Cds3/LConn1 -- P2/RConn1 -- MOSFETA1/RConn2 -- Cds/RConn1 -- MOSFETA2/RConn1
  Simulink-PS Converter4/RConn1 -- MOSFETA1/LConn1
  Thermal Resistor/LConn1 -- Temperature Source/LConn1
  Thermal Resistor/RConn1 -- MOSFETA1/LConn2
  Cds2/LConn1 -- MOSFETB2/RConn1 -- N2/RConn1 -- MOSFETB1/RConn2 -- Cds1/RConn1
  Thermal Resistor1/RConn1 -- MOSFETB1/LConn2
  Simulink-PS Converter2/RConn1 -- MOSFETB1/LConn1
  Thermal Resistor1/LConn1 -- Temperature Source1/LConn1
  Thermal Resistor2/RConn1 -- MOSFETB2/LConn2
  Simulink-PS Converter3/RConn1 -- MOSFETB2/LConn1
  Thermal Resistor2/LConn1 -- Temperature Source2/LConn1
  Thermal Resistor3/RConn1 -- MOSFETA2/LConn2
  Simulink-PS Converter1/RConn1 -- MOSFETA2/LConn1
  Thermal Resistor3/LConn1 -- Temperature Source3/LConn1
  Cds2/RConn1 -- Cds3/RConn1 -- N1/RConn1 -- MOSFETA2/RConn2 -- MOSFETB2/RConn2

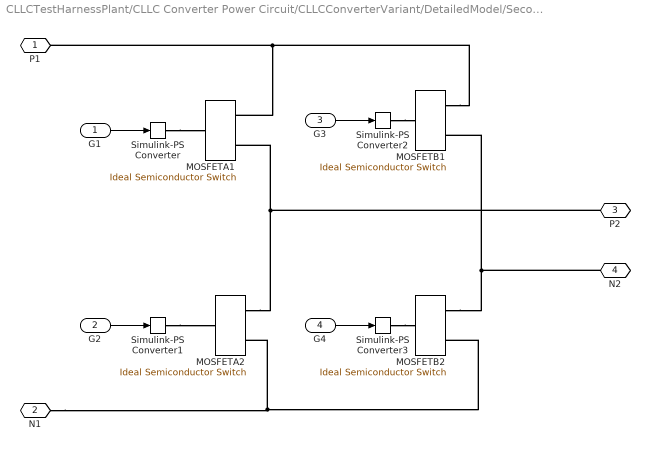
== system CLLCTestHarnessPlant/CLLC Converter Power Circuit/CLLCConverterVariant/DetailedModel/Secondary Converter/Secondary Converter Full Bridge/Ideal Switch ==
  G1 : Inport
  G2 : Inport  Port=2
  G3 : Inport  Port=3
  G4 : Inport  Port=4
  MOSFETA1 : ee_lib/Semiconductors & Converters/Ideal Semiconductor Switch  port_option=ee.enum.controlport.ps  Ron=SecondaryRon Ohm  Goff=SecondaryGoff 1/Ohm  Vth=SecondaryVth V  diode_param=ee.enum.semiconductors.protectionDiode.nodynamics  diode_Vf=SecondaryVbodydiodeOn V  diode_Ron=SecondaryRbodydiodeOn Ohm  diode_Goff=SecondaryGbodydiodeOff 1/Ohm  diode_C=50e-9 F  diode_iRM=-235 A  diode_iF=300 A  diode_idot=-50 A/us  diode_trr_param=ee.enum.converters.diodetrr.trr_factor  diode_trr_factor=3  diode_trr=15 us  diode_Qrr=1500 s*uA
  MOSFETA2 : ee_lib/Semiconductors & Converters/Ideal Semiconductor Switch  port_option=ee.enum.controlport.ps  Ron=SecondaryRon Ohm  Goff=SecondaryGoff 1/Ohm  Vth=SecondaryVth V  diode_param=ee.enum.semiconductors.protectionDiode.nodynamics  diode_Vf=SecondaryVbodydiodeOn V  diode_Ron=SecondaryRbodydiodeOn Ohm  diode_Goff=SecondaryGbodydiodeOff 1/Ohm  diode_C=50e-9 F  diode_iRM=-235 A  diode_iF=300 A  diode_idot=-50 A/us  diode_trr_param=ee.enum.converters.diodetrr.trr_factor  diode_trr_factor=3  diode_trr=15 us  diode_Qrr=1500 s*uA
  MOSFETB1 : ee_lib/Semiconductors & Converters/Ideal Semiconductor Switch  port_option=ee.enum.controlport.ps  Ron=SecondaryRon Ohm  Goff=SecondaryGoff 1/Ohm  Vth=SecondaryVth V  diode_param=ee.enum.semiconductors.protectionDiode.nodynamics  diode_Vf=SecondaryVbodydiodeOn V  diode_Ron=SecondaryRbodydiodeOn Ohm  diode_Goff=SecondaryGbodydiodeOff 1/Ohm  diode_C=50e-9 F  diode_iRM=-235 A  diode_iF=300 A  diode_idot=-50 A/us  diode_trr_param=ee.enum.converters.diodetrr.trr_factor  diode_trr_factor=3  diode_trr=15 us  diode_Qrr=1500 s*uA
  MOSFETB2 : ee_lib/Semiconductors & Converters/Ideal Semiconductor Switch  port_option=ee.enum.controlport.ps  Ron=SecondaryRon Ohm  Goff=SecondaryGoff 1/Ohm  Vth=SecondaryVth V  diode_param=ee.enum.semiconductors.protectionDiode.nodynamics  diode_Vf=SecondaryVbodydiodeOn V  diode_Ron=SecondaryRbodydiodeOn Ohm  diode_Goff=SecondaryGbodydiodeOff 1/Ohm  diode_C=50e-9 F  diode_iRM=-235 A  diode_iF=300 A  diode_idot=-50 A/us  diode_trr_param=ee.enum.converters.diodetrr.trr_factor  diode_trr_factor=3  diode_trr=15 us  diode_Qrr=1500 s*uA
  Simulink-PS Converter{,1..3} (4 alike) : nesl_utility/Simulink-PS Converter  PhysicalDomain=network_engine_domain  SubClassName=ps_input  LeftPortType=input  RightPortType=output  PseudoPeriodic=off  Frequencies=[]  NoiseDistribution=none  NoiseParameters=[]  Unit=1  AffineConversion=off  FilteringAndDerivatives=provide  SimscapeFilterOrder=1  InputFilterTimeConstant=0.001  UdotUserProvided=0
  P1 : PMIOPort  Side=Right
  N1 : PMIOPort  Port=2  Side=Right
  P2 : PMIOPort  Port=3  Side=Left
  N2 : PMIOPort  Port=4  Side=Left
  wires:
  G1/1 -> Simulink-PS Converter/1
  G2/1 -> Simulink-PS Converter1/1
  G3/1 -> Simulink-PS Converter2/1
  G4/1 -> Simulink-PS Converter3/1
  connections:
  N2/RConn1 -- MOSFETB2/RConn1 -- MOSFETB1/RConn2
  P2/RConn1 -- MOSFETA2/RConn1 -- MOSFETA1/RConn2
  P1/RConn1 -- MOSFETB1/RConn1 -- MOSFETA1/RConn1
  N1/RConn1 -- MOSFETB2/RConn2 -- MOSFETA2/RConn2
  Simulink-PS Converter/RConn1 -- MOSFETA1/LConn1
  Simulink-PS Converter1/RConn1 -- MOSFETA2/LConn1
  Simulink-PS Converter2/RConn1 -- MOSFETB1/LConn1
  Simulink-PS Converter3/RConn1 -- MOSFETB2/LConn1
